simulink model "ev_powertrain"  (R2025b)
settings: Solver=ode3  StartTime=0  StopTime=589  FixedStep=0.01  RelTol=1e-3
PreLoadFcn:
  | init_params
values from neighbouring files (symbols this model uses):
  ekfb = batt    [init_params.m]    (also in make_plots.m; run_tests.m)
  veh = struct('m',1500,'Cd',0.28,'A',2.2,'Crr',0.015,'rho',1.225,               'g',9.81,'rw',0.30,'Fmax',6000)    [init_params.m]
undefined symbols (not defined in the file or in its folder): batt, ekf, magnitude
libraries: autolibshared x2
settings Model: Creator=samar  LastModifiedBy=samar

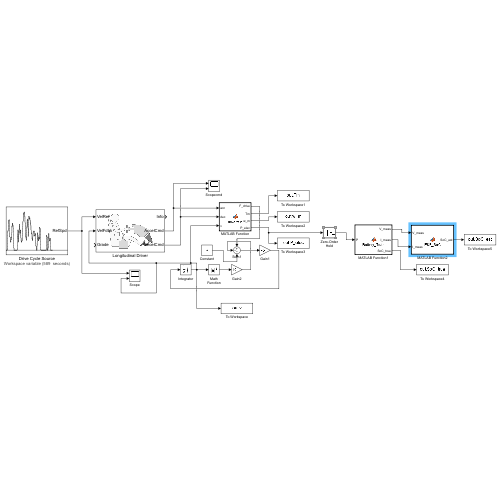
[thumbnail: Simulink's stored preview of the top-level diagram]
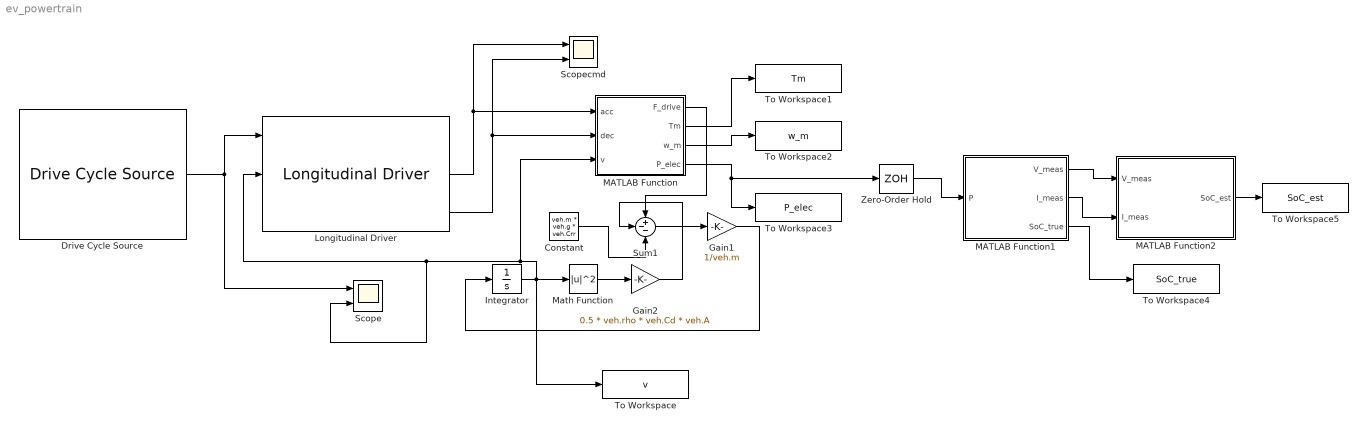
== system ev_powertrain ==
  Constant : Constant  Value=veh.m * veh.g * veh.Crr
  Drive Cycle Source : autolibshared/Drive Cycle Source  cycleVar=Workspace variable  wsVar=wltp_data  fileVar=cycleFTP75.mat  tfinal="589  seconds"  cycleRepeat=off  outAccPort=off  outGearPort=off  gearList=No gear data  t_wot1=5  xdot_woto=0  xdot_wot1=30  t_wot2=20  xdot_wot2=0  t_wotend=30  srcUnit=m/s  outUnit=m/s  srcAccUnit=m/s/s  outAccUnit=m/s^2  dt=0  aMode=1  faultOption=off  velBnd=2  velBndUnit=mph  inUnit=m/s  timeBnd=1  failOption=off  stopSim=off  maxFaultCnt=10  maxFaultTime=2  maxTotFaultTime=15  traceOption=off  dtTrace=1  traceWindow=10  lastDCname=Custom Data Set  lastOutUnit=mph  lastDT=0  lastTB=1  lastSB=2  forceCalcBound=off
  Gain1 : Gain  Gain=1/veh.m
  Gain2 : Gain  Gain=0.5 * veh.rho * veh.Cd * veh.A
  Integrator : Integrator  LimitOutput=on  LowerSaturationLimit=0
  Longitudinal Driver : autolibshared/Longitudinal Driver  extAccelOvr=off  extDecelOvr=off  extAccelHld=off  extDecelHld=off  extAccelZero=off  extDecelZero=off  cntrlType=PI  shftType=None  velUnits=m/s  gearOut=off  Kp=35  Ki=5  Kff=.1  Kg=.01  VehVelVec=[0 100]  KffVec=[.1 .1]  KpVec=[10 10]  KiVec=[5 5]  KgVec=[0 0]  m=1500  Kpt=3000  tau=.1  L=2  aR=200  bR=2.5  cR=.5  g=9.81  vnom=100  Kaw=.1  tauerr=.03  tauPt=2  GearInit=0  tShift=.1  pdlVec=[0.1 0.4 0.5 0.9]  upShftTbl=[-1 12.9375 26.4375 39.9375 51.18749999999999 62.4375 72.84375 83.25;-1 16.3125 29.8125 43.3125 54.5624 65.8125 76.78125 87.75;-1 19.6875 33.1875 46.68749999999999 57.9375 69.1875 80.71875 92.25;-1 33 52.5 77.25 100.5 138.75 161.875 185]  dwnShftTbl=[1 9.5625 23.0625 36.5625 47.8125 59.0625 68.90625 78.75;1 12.9375 26.4375 39.9375 51.18749999999999 62.4375 72.84375 83.25;1 16.3125 29.8125 43.3125 54.562499 65.8125 76.78125 87.75;1 19.6875 33.1875 46.68749999999999 57.9375 69.1875 80.71875 92.25]  tClutch=.5  tRev=.5  tPark=120  aMode=1  UpGearVec="[0  1  2  3  4  5  6  7]"  DownGearVec="[1  2  3  4  5  6  7  8]"
  MATLAB Function : MATLAB Function  TreatAsAtomicUnit=on
  MATLAB Function1 : MATLAB Function  TreatAsAtomicUnit=on
  MATLAB Function2 : MATLAB Function  TreatAsAtomicUnit=on
  Math Function : Math  Operator=magnitude^2
  Scope : Scope  NumInputPorts=2
      settings: ActiveDisplayYMinimum=-4.7826770641607368  ActiveDisplayYMaximum=19.136099563747017
  Scopecmd : Scope  NumInputPorts=2
      settings: ActiveDisplayYMinimum=-0.21251727628698014  ActiveDisplayYMaximum=0.8075572899343525
  Sum1 : Sum  Inputs=+--
  To Workspace : ToWorkspace  VariableName=v  SampleTime=-1
  To Workspace1 : ToWorkspace  VariableName=Tm  SaveFormat=Timeseries  SampleTime=-1
  To Workspace2 : ToWorkspace  VariableName=w_m  SaveFormat=Timeseries  SampleTime=-1
  To Workspace3 : ToWorkspace  VariableName=P_elec  SaveFormat=Timeseries  SampleTime=-1
  To Workspace4 : ToWorkspace  VariableName=SoC_true  SaveFormat=Timeseries  SampleTime=-1
  To Workspace5 : ToWorkspace  VariableName=SoC_est  SaveFormat=Timeseries  SampleTime=-1
  Zero-Order Hold : ZeroOrderHold  SampleTime=batt.Ts
  wires:
  Drive Cycle Source/1 -> Longitudinal Driver/1, Scope/1
  Longitudinal Driver/2 -> MATLAB Function/1(acc), Scopecmd/1
  Longitudinal Driver/3 -> MATLAB Function/2(dec), Scopecmd/2
  Sum1/1 -> Gain1/1
  Math Function/1 -> Gain2/1
  Gain2/1 -> Sum1/2
  Constant/1 -> Sum1/3
  Integrator/1 -> To Workspace/1, MATLAB Function/3(v), Scope/2, Longitudinal Driver/2, Math Function/1
  Gain1/1 -> Integrator/1
  MATLAB Function/1(F_drive) -> Sum1/1
  MATLAB Function/2(Tm) -> To Workspace1/1
  MATLAB Function/3(w_m) -> To Workspace2/1
  MATLAB Function/4(P_elec) -> Zero-Order Hold/1, To Workspace3/1
  Zero-Order Hold/1 -> MATLAB Function1/1(P)
  MATLAB Function1/1(V_meas) -> MATLAB Function2/1(V_meas)
  MATLAB Function1/2(I_meas) -> MATLAB Function2/2(I_meas)
  MATLAB Function1/3(SoC_true) -> To Workspace4/1
  MATLAB Function2/1(SoC_est) -> To Workspace5/1

== matlab function ev_powertrain/MATLAB Function1 ==
  data: P input; V_meas output; I_meas output; SoC_true output; batt parameter
function [V_meas, I_meas, SoC_true] = Battery_Truth(P, batt)
persistent soc v1
if isempty(soc)
    soc = batt.SoC_init;  v1 = 0;
end
dt  = batt.Ts;
ocv = interp1(batt.soc_lut, batt.ocv_lut, soc, 'linear', 'extrap');
Vx  = ocv - v1;
I   = (Vx - sqrt(max(Vx^2 - 4*batt.R0*P, 0))) / (2*batt.R0);  % A, + = discharge
Vt  = Vx - I*batt.R0;

V_meas   = Vt + 0.1*randn;      % 0.1 V sensor noise (matches ekf.R = 1e-2)
I_meas   = I  + 0.5*randn;      % 0.5 A sensor noise
SoC_true = soc;

soc = min(max(soc - I*dt/(batt.Capacity_Ah*3600), 0), 1);
v1  = v1 + dt*(-v1/(batt.R1*batt.C1) + I/batt.C1);
end

== matlab function ev_powertrain/MATLAB Function ==
  data: acc input; F_drive output; dec input; v input; Tm output; w_m output; P_elec output; drv parameter
function [F_drive, Tm, w_m, P_elec] = drivetrain(acc, dec, v, drv)
% Inputs : acc, dec (0..1 from driver), v (m/s), drv (parameter struct)
% Outputs: F_drive (N at wheels), Tm (Nm), w_m (rad/s), P_elec (W)

w_m    = max(v,0)/drv.rw*drv.G;                 % Motor speed
Tlim   = min(drv.Tmax, drv.Pmax/max(w_m,1));    % Torque limit envelope
T_trac = acc*Tlim;                            % Traction torque
F_bd   = dec*drv.Fbrake;                      % Total brake demand
fade   = min(max(v/2,0),1);                   % Fade regen below 2 m/s
T_reg  = min(F_bd*drv.rw/drv.G, Tlim)*fade;   % Regen torque
Tm     = T_trac - T_reg;                      % Net motor torque
F_fric = F_bd - T_reg*drv.G/drv.rw;          % Mechanical friction brake force
F_drive = Tm*drv.G/drv.rw - F_fric;           % Net tractive force

P_mech = Tm*w_m;
P_loss = drv.kc*Tm^2 + drv.ki*w_m + drv.kw*w_m^3 + drv.P0*(w_m>1);
P_elec = P_mech + P_loss;                     % Electrical power (+ discharge, - charge)
end

== matlab function ev_powertrain/MATLAB Function2 ==
  data: V_meas input; SoC_est output; I_meas input; ekfb parameter; ekf parameter
function SoC_est = EKF_SoC(V_meas, I_meas, ekfb, ekf)
persistent x P
if isempty(x)
    x = [ekf.SoC0; 0];  P = ekf.P0;
end
dt = ekfb.Ts;
a  = exp(-dt/(ekfb.R1*ekfb.C1));

% ---- correct (using this step's measurement) ----
s    = x(1);
ocv  = interp1(ekfb.soc_lut, ekfb.ocv_lut, s, 'linear', 'extrap');
d    = 1e-3;
docv = (interp1(ekfb.soc_lut, ekfb.ocv_lut, s+d, 'linear', 'extrap') - ...
        interp1(ekfb.soc_lut, ekfb.ocv_lut, s-d, 'linear', 'extrap')) / (2*d);
yhat = ocv - x(2) - I_meas*ekfb.R0;
H    = [docv, -1];
S    = H*P*H' + ekf.R;
K    = (P*H') / S;
x    = x + K*(V_meas - yhat);
P    = (eye(2) - K*H)*P;
x(1) = min(max(x(1), 0), 1);
SoC_est = x(1);

% ---- predict (next step) ----
x = [x(1) - I_meas*dt/(ekfb.Capacity_Ah*3600);
     a*x(2) + ekfb.R1*(1-a)*I_meas];
F = [1 0; 0 a];
P = F*P*F' + ekf.Q;
end
